simulink model "BimanualCarvingModifiedSnapshot"  (R2013a)
settings: Solver=ode4  SolverMode=SingleTasking  StartTime=0.0  StopTime=inf  FixedStep=0.0005  RelTol=1e-3
StartFcn:
  |  warndlg('Dexterit-E models cannot run under simulation. Please compile your model and run it from within Dexterit-E.');set_param(bdroot,'SimulationCommand','stop')
model workspace (MAT data in the model file):
  BKIN_STEP_TIME = 0.0005
  col_x = 1
  col_y = 2
  WIDTH = 3
  HEIGHT = 4
  TARGET_COL = 1
  LOAD = 2
  TRAJ_DURATION_COL = 3
  MAX_LOAD = 2
  FORCE_ON = 1
  HAND_RADIUS = 6
  REST_COL = 4
  TRAINING_COL = 5
  HAND_COLOR = 5
  TARGET_STROKE = 8
  TARGET_RADIUS = 9
  xMaxCursor = 15
  yMaxCursor = 16
  TARGET_COLOR = 7
  START_X = 10
  START_Y = 11
  STIFFNESS_MATERIAL = 3
  MATERIAL_MASS = 4
  MATERIAL_DAMPING = 5
  STIFFNESS_HANDS = 6
  MATERIAL_GOAL_COLOR = 12
  SCALE_VIBRATION = 7
  STONE_WIDTH = 6
  MATERIAL_DUCTILITY = 8
  TARG_COLOR = 1
  TEXT_COLOR = 13
  TEXTBOX_WIDTH = 14
  TEXTBOX_HEIGHT = 15
  ROTATION = 16
  LABEL_TEXT = 17
  LABEL_COLOR = 18
  LABEL_HEIGHT = 19
  ADVANCE_EMG_PLACEMENT = 2
  ADVANCE_EMG_MAX = 3
  EMG_ADVANCE_BUTTON = 1
  EMG_MVC_BUTTON = 2
  START_TRIAL = 3
  END_TRIAL = 4
  MUSC_NUM = 2
  HAND_DISTANCE = 3
  SYN_NUM = 4
undefined symbols (not defined in the file or in its folder): slselsubs
libraries: xpclib x9, simulink x6, General x3, KINARM_loads x2, Video x2, KINARM_IO x1, KINARM_EP_loads x1
(part 6 of 6)

== matlab function BimanualCarvingModifiedSnapshot/MATLAB Function ==
  data: resid output; emg input; syn_num input
function resid  = emg_similarity(emg,syn_num)
%#codegen

persistent C;

if isempty(C)
    switch syn_num
        case 6
            C = master_synergies_6();
        case 7
            C = master_synergies_7();
        case 8
            C = master_synergies_8();
        case 9
            C = master_synergies_9();
        case 10
            C = master_synergies_10();
        case 11
            C = master_synergies_11();
        case 12
            C = master_synergies_12();
        case 13
            C = master_synergies_13();
        case 14
            C = master_synergies_14();
        case 15
            C = master_synergies_15(); 
        case 16
            C = master_synergies_16();
        otherwise
            C = master_synergies_7();
    end
end

d = emg(1:end,1);

n = size(C,2);
% Initialize vector of n zeros and Infs (to be used later)
nZeros = zeros(n,1);
wz = nZeros;

% Initialize set of non-active columns to null
P = false(n,1);
% Initialize set of active columns to all and the initial point to zeros
Z = true(n,1);
x = nZeros;

resid = d - C*x;
w = C'*resid;

% Set up iteration criterion
outeriter = 0;
iter = 0;
itmax = 3*n;

tol = 10*eps*norm(C,1)*length(C);

% Outer loop to put variables into set to hold positive coefficients
while any(Z) && any(w(Z) > tol)
    outeriter = outeriter + 1;
    % Reset intermediate solution z
    z = nZeros;
    % Create wz, a Lagrange multiplier vector of variables in the zero set.
    % wz must have the same size as w to preserve the correct indices, so
    % set multipliers to -Inf for variables outside of the zero set.
    wz(P) = -Inf;
    wz(Z) = w(Z);
    % Find variable with largest Lagrange multiplier
    [~,t] = max(wz);
    % Move variable t from zero set to positive set
    P(t) = true;
    Z(t) = false;
    % Compute intermediate solution using only variables in positive set
    z(P) = C(:,P)\d;
    % inner loop to remove elements from the positive set which no longer belong
    while any(z(P) <= 0)
        iter = iter + 1;
        if iter > itmax
            %            msg = getString(message('MATLAB:lsqnonneg:IterationCountExceeded'));
            %            if verbosity
            %                disp(msg)
            %            end
            %            exitflag = 0;
            %            output.iterations = outeriter;
            %            output.message = msg;
            %            output.algorithm = 'active-set';
            resnorm = sum(resid.*resid);
            x = z;
            lambda = w;
            return
        end
        % Find indices where intermediate solution z is approximately negative
        Q = (z <= 0) & P;
        % Choose new x subject to keeping new x nonnegative
        alpha = min(x(Q)./(x(Q) - z(Q)));
        x = x + alpha*(z - x);
        % Reset Z and P given intermediate values of x
        Z = ((abs(x) < tol) & P) | Z;
        P = ~Z;
        z = nZeros;           % Reset z
        z(P) = C(:,P)\d;      % Re-solve for z
    end
    x = z;
    resid = d - C*x;
    w = C'*resid;
end
end

function C = master_synergies_6()

C = [ 0.6059         0    0.0982    0.3257    0.0587    0.0562;
    0.3321    0.1853    0.0774    0.0907    0.3019    0.1813;
    0.1383    0.6018         0    0.1365         0    0.2733;
    0    0.0039    0.4293    0.0680    0.2207         0;
    0.1053    0.4074         0         0         0    0.2375;
    0.1749         0    0.7674    0.1333    0.0094    0.1202;
    0.2135    0.4062         0    0.0447    0.0003    0.0525;
    0.3188         0    0.2392    0.0240    0.3338         0;
    0.2886         0         0    0.5969    0.0171    0.3358;
    0.0632    0.0389    0.0341    0.0191    0.2286    0.4584;
    0.2456    0.0036    0.3484    0.4769    0.6912         0;
    0.0068    0.4849    0.0629    0.3820    0.1736    0.1716;
    0.1126    0.0665    0.1033    0.2344    0.4184    0.0828;
    0    0.0880         0    0.1599         0    0.5841;
    0.2590    0.1541    0.1131    0.1704         0    0.1773;
    0.2953    0.0010    0.0630    0.0508    0.0982    0.2895];
end

function C = master_synergies_7()

C = [0.2361    0.5046    0.0063    0.0514    0.0762    0.1018    0.5583;
    0.0626    0.6381    0.2251    0.0416    0.0042    0.3024    0.1665;
    0.0099    0.1110    0.0041    0.5932    0.0038    0.2818    0.0222;
    0.3413         0    0.3384         0    0.0118         0    0.0002;
    0    0.1591         0    0.3446         0    0.2055         0;
    0.8267    0.0618    0.2096    0.0154    0.0543    0.1097    0.0277;
    0.0486    0.0867         0    0.4538    0.2466         0    0.0104;
    0.2047    0.3779    0.3780         0    0.1608         0    0.0902;
    0.0667    0.0003    0.0100    0.1339    0.1139    0.4125    0.5722;
    0    0.0064    0.0628         0    0.6909    0.2578         0;
    0.2141    0.2612    0.6779    0.0381    0.1927    0.1565    0.4705;
    0.0114    0.0040    0.2441    0.5000    0.0084    0.3172    0.1190;
    0.0198    0.1710    0.3527    0.0473    0.1981    0.1708    0.2149;
    0.0064    0.0110    0.0010    0.0279    0.0479    0.5863         0;
    0.1867    0.0999    0.0025    0.2151    0.2154    0.1211    0.1699;
    0.1015    0.1971    0.0198    0.0118    0.5375    0.1232    0.1141];

end

function C = master_synergies_8()

C = [ 0.4473    0.3964    0.1653    0.0355    0.1020    0.5229    0.0261    0.0115;
    0.0285    0.7249    0.0686    0.0500    0.0628    0.2279    0.0889    0.3301;
    0.0517    0.0993    0.1484    0.6898    0.3641    0.0000    0.0003    0.0000;
    0.0250    0.0000    0.0000    0.0000    0.0000    0.0867    0.4422    0.1256;
    0.0000    0.1156    0.0027    0.4693    0.2537    0.0006    0.0000    0.0081;
    0.0285    0.0118    0.0145    0.0000    0.1628    0.3434    0.7008    0.0000;
    0.0281    0.0338    0.4232    0.4431    0.0439    0.1244    0.0000    0.0362;
    0.1715    0.0510    0.0000    0.0856    0.0000    0.5682    0.1402    0.2302;
    0.5959    0.0444    0.1387    0.0688    0.5056    0.0768    0.0286    0.0373;
    0.0052    0.0000    0.0548    0.0259    0.2395    0.0613    0.0407    0.5230;
    0.5523    0.3729    0.0916    0.0230    0.0091    0.0773    0.4871    0.5104;
    0.0226    0.2717    0.8393    0.1750    0.2185    0.0406    0.0678    0.1765;
    0.2321    0.2706    0.0940    0.0305    0.0456    0.0082    0.1862    0.3985;
    0.0000    0.0440    0.0002    0.0000    0.5584    0.0000    0.0000    0.1577;
    0.1892    0.0177    0.1459    0.2290    0.2196    0.2362    0.0772    0.0182;
    0.1200    0.0002    0.0386    0.0810    0.1930    0.3711    0.0000    0.2650];

end

function C = master_synergies_9()

C = [0.4154    0.1071    0.1031    0.5616         0    0.0589    0.1282         0    0.1961;
    0.2289    0.0221    0.0624    0.6351    0.0007         0    0.3077    0.2958         0;
    0.0457         0    0.3796    0.1022    0.7570    0.2097    0.0499         0         0;
    0.0908    0.4127         0         0         0    0.0101    0.1940    0.0988         0;
    0         0    0.2481    0.0969    0.5721         0    0.1394    0.0069         0;
    0.0770    0.8327    0.0579    0.1964         0         0    0.0150    0.0748    0.1636;
    0         0    0.0124    0.2192    0.2617    0.4170         0         0    0.4660;
    0.1660    0.1223         0    0.2036         0         0    0.6855         0    0.1629;
    0.4004         0    0.5906    0.0466    0.0589    0.1919    0.1056         0         0;
    0.0041         0    0.0842         0    0.0131         0    0.0481    0.6103    0.5818;
    0.6728    0.3045    0.0577    0.1792         0    0.0962    0.2672    0.4640         0;
    0.0379         0    0.3971    0.1856         0    0.8413    0.3095    0.0652         0;
    0.3270    0.0679    0.0566    0.1250    0.0255    0.0633    0.1523    0.3976    0.0374;
    0         0    0.4330    0.1048    0.0002    0.0136    0.0168    0.3790         0;
    0.0968    0.1093    0.2007    0.1583    0.1635    0.1432    0.0970         0    0.2817;
    0.0220         0    0.1686    0.1138    0.0077         0    0.3817    0.0579    0.5213];
end

function C = master_synergies_10()

C = [0.4986    0.1733    0.0367    0.4603    0.1482         0    0.0499    0.0111    0.0009         0;
    0.5610    0.0771    0.2267         0    0.0812    0.0400         0    0.5313         0         0;
    0         0    0.6666    0.1875    0.1703         0         0    0.1027    0.5281    0.1122;
    0    0.3723         0         0         0    0.2823         0         0    0.0324    0.3422;
    0.0393         0    0.5953    0.0003    0.0925         0    0.1203    0.0059    0.1207    0.0717;
    0    0.8366    0.0060    0.0965    0.0166    0.2299    0.0212    0.0633    0.0647    0.2363;
    0.0961         0    0.1922    0.0963    0.1991         0    0.0015    0.0222    0.7730    0.0491;
    0.4351    0.0715         0         0         0    0.0157    0.0037    0.0915         0    0.7138;
    0.0336         0    0.0213    0.7040    0.2206    0.1786    0.2542    0.1029         0    0.2509;
    0         0         0    0.0018         0    0.2589    0.6350    0.2435    0.1760    0.0651;
    0.3789    0.3157         0    0.3611    0.1261    0.7676    0.1259         0    0.0010    0.1354;
    0.1213         0    0.2816    0.0028    0.8945         0    0.3734    0.0095         0    0.1218;
    0.2207    0.0857    0.0583    0.1355    0.1095    0.4212    0.2106    0.0735         0         0;
    0         0    0.0758    0.0610    0.0479    0.0076    0.1904    0.7866    0.0100    0.0738;
    0.0641    0.1157    0.1403    0.2653    0.1074    0.0026    0.1498         0    0.2697    0.2213;
    0.1560         0    0.0542    0.1260    0.0596         0    0.5065         0         0    0.3776];

end

function C = master_synergies_11()

C = [ 0.6267         0         0    0.3526         0    0.5868         0    0.0290         0    0.0100         0;
    0.0928         0    0.2848    0.7848         0    0.2838         0         0    0.1110         0         0;
    0.0727    0.7087    0.0213    0.0284         0    0.0469    0.1440         0    0.2549    0.4188         0;
    0         0    0.3660         0    0.3437         0         0    0.0812    0.0430    0.0288    0.0164;
    0    0.5699         0    0.0503    0.0029    0.1112         0    0.0926    0.1385         0    0.0129;
    0.2034         0    0.1110    0.1557    0.9149    0.0419    0.0453    0.1059    0.0242    0.0716         0;
    0.0633    0.2088         0    0.1548         0    0.1978         0         0    0.0780    0.8336    0.1164;
    0         0    0.5202    0.0670         0    0.5700         0         0    0.2355    0.0045    0.0189;
    0.4181    0.0649    0.0571    0.0372         0         0    0.3762    0.0922    0.6754         0         0;
    0.0004         0         0         0    0.0498    0.1478    0.3393    0.6502    0.0067    0.2170         0;
    0.5158         0    0.6441    0.2784    0.0183    0.1438         0    0.4946         0         0         0;
    0.1802    0.3229         0    0.2333         0    0.1151    0.2538         0         0         0    0.9915;
    0.2333    0.0377    0.2887    0.2184         0    0.0854    0.0204    0.3955         0         0    0.0446;
    0    0.0579    0.0068    0.0512    0.0187         0    0.8089         0    0.1247    0.0439    0.0094;
    0.1421    0.1273         0    0.1116    0.1612    0.1440    0.0371    0.0738    0.3545    0.2731         0;
    0         0         0    0.0872    0.1255    0.3331         0    0.3674    0.4921    0.0055    0.0246];

end

function C = master_synergies_12()

C = [ 0.7011         0    0.1260         0    0.4795         0    0.0246    0.1420         0         0    0.2258       0;
    0.2721         0    0.0341         0    0.3797    0.2816    0.5681    0.2077         0         0         0    0.3002;
    0         0    0.2804         0    0.0110    0.3023         0    0.4993    0.1884    0.2485    0.0360    0.9492;
    0    0.4017         0    0.4368    0.0518         0    0.0317         0         0         0         0         0;
    0    0.0125    0.1436         0         0    0.1829         0    0.7672    0.0852    0.1739    0.0414    0.0511;
    0.1513    0.8869         0    0.2600    0.0407    0.0063    0.0048         0    0.0045    0.0497    0.1281    0.0421;
    0.0491         0    0.7884         0    0.0348    0.0997         0    0.0379    0.0678    0.2205    0.0185    0.0169;
    0.1555         0         0    0.4127    0.6706         0    0.0501    0.0471    0.0002         0    0.0063         0;
    0.2981         0    0.0862    0.1803    0.0589    0.4909    0.0959         0    0.0596    0.5564         0    0.0600;
    0.0326         0    0.0000    0.0327    0.0957         0    0.2165         0         0    0.1787    0.8417         0;
    0.4802    0.1772    0.0091    0.6794    0.2152         0    0.5173    0.0512    0.0034         0    0.2337         0;
    0    0.0120    0.3977         0    0.0096    0.2549    0.2803    0.2526    0.9724         0    0.0483    0.0023;
    0.2241    0.0102         0    0.2667    0.1009    0.0233    0.4269    0.1000    0.0537    0.0253    0.2408    0.0237;
    0    0.0279    0.0178    0.0066         0    0.6702         0    0.0787    0.0074    0.0318    0.2909         0;
    0.1181    0.1386    0.3100    0.0703    0.0903    0.1730    0.0262    0.1014         0    0.3897         0         0;
    0.0119    0.0145         0         0    0.3052    0.0156    0.2964    0.0471    0.0229    0.6015    0.1454         0];

end

function C = master_synergies_13()

C = [0.4192    0.0916         0         0         0    0.0643    0.3018    0.9064         0         0    0.1337    0.0079         0;
    0.3740    0.1303         0    0.1148         0         0    0.0495         0    0.2485         0    0.9012         0    0.0689;
    0.0322    0.7385         0    0.1716    0.3918    0.1511    0.1826         0    0.0703         0         0         0    0.1042;
    0.0513         0    0.3098    0.0162         0    0.0250    0.2180    0.0287         0    0.4563    0.1158         0    0.0011;
    0    0.5836         0         0         0         0    0.0697    0.0258    0.2212         0    0.1315    0.2304    0.1023;
    0.2294         0    0.9350    0.0655    0.0864    0.1329    0.0127    0.1139         0    0.0007    0.0609         0    0.0907;
    0.0489    0.2372         0         0    0.7054         0    0.2310    0.1142         0         0    0.1122    0.1288    0.0107;
    0.3397         0         0         0         0    0.0715    0.7998    0.1187    0.0394         0         0    0.0459    0.1225;
    0.1882    0.0494         0    0.3749    0.1292    0.7747    0.0972    0.0989         0         0    0.1000         0    0.0593;
    0.0007         0    0.0600    0.1048    0.0239    0.0557    0.0621    0.0192         0         0    0.1753    0.3761    0.8602;
    0.5917         0    0.1283    0.0382    0.0683    0.3674    0.0732    0.2509         0    0.7505         0         0    0.3835;
    0.0010         0    0.0467    0.3337    0.5202    0.3822         0    0.1442    0.9369         0         0    0.0102         0;
    0.2740    0.0167         0    0.0743    0.0172    0.1146         0    0.1462    0.0711    0.4782    0.1199    0.1512    0.2451;
    0    0.0189    0.0160    0.8255    0.0421    0.0019    0.0789         0    0.0051         0    0.0309    0.0256         0;
    0.0777    0.1713    0.0859    0.0264    0.2161    0.2037    0.2027    0.1422         0         0    0.2586    0.2396         0;
    0.2087         0         0    0.0272    0.0044    0.1032    0.2481    0.0356         0         0         0    0.8400         0];

end

function C = master_synergies_14()

C = [0.0658    0.8315    0.3623    0.3054    0.0918         0    0.0154         0         0    0.1063         0         0         0    0.0079;
    0.0038    0.3625         0    0.1597    0.8230         0         0    0.1820         0         0         0         0    0.1647    0.1061;
    0    0.0541    0.2498    0.1010    0.0496         0    0.1656    0.5613    0.8729    0.0257    0.1291         0         0    0.0075;
    0.1531    0.0414    0.0043    0.0970    0.0583    0.1241         0         0         0    0.0125    0.0395         0    0.8465    0.0420;
    0         0    0.1842         0         0         0    0.0825    0.7553    0.1601    0.0338    0.0950    0.1002         0    0.0899;
    0.1360    0.0882    0.1645    0.1577    0.0862    0.9568         0         0         0         0         0         0    0.4057    0.1042;
    0    0.1579    0.1105    0.1048         0         0         0    0.1761    0.3970    0.0331    0.0056         0         0    0.9063;
    0.0668    0.2608         0    0.6901    0.1444    0.0418         0         0         0    0.1791         0         0    0.1005         0;
    0.2427    0.0194    0.7816    0.2601    0.1676         0    0.0265         0         0    0.1390    0.0530         0         0    0.0048;
    0.0105         0         0    0.1403    0.1383    0.0058    0.0034    0.0184    0.0012    0.1897    0.1011    0.9044         0    0.0034;
    0.8485    0.1839    0.1112    0.4146    0.3034    0.2377         0         0         0    0.2042    0.1958         0         0    0.0351;
    0.0438    0.0806    0.0721    0.1096         0         0    0.9805    0.1726    0.1986    0.1481         0    0.3109         0    0.2030;
    0.4103    0.1052         0    0.1103    0.2762         0    0.0534    0.0558    0.0098    0.2449    0.1476    0.1096    0.0880         0;
    0         0    0.0426    0.0213    0.1013         0    0.0247    0.0316    0.0256    0.0593    0.9484    0.2518    0.0582    0.0128;
    0    0.1418    0.3207    0.1245    0.0900    0.0485         0    0.1266    0.1211    0.1976         0         0    0.2632    0.3220;
    0.0021    0.0079    0.0009    0.2240    0.2149    0.0923    0.0058         0         0    0.8556    0.0127         0    0.0364    0.0132];

end

function C = master_synergies_15()

C = [ 0.4462    0.7696         0    0.2903         0         0    0.0693         0         0    0.0006         0         0    0.0000    0.0118         0;
    0.3767    0.3395         0         0    0.0120         0         0    0.0207    0.0371    0.9074         0         0         0    0.2974         0;
    0    0.0040    0.8797         0         0    0.1721    0.3340         0    0.2984    0.1297    0.0427    0.1668         0         0         0;
    0.1327         0         0    0.2290    0.1006         0    0.0137         0    0.1129    0.0016         0         0    0.0679         0    0.9196;
    0    0.0073    0.2200         0         0    0.0807    0.0798    0.0457    0.1362    0.0635    0.0912    0.9854    0.0051    0.0026         0;
    0.1486         0         0    0.8910    0.1577    0.0458    0.0438    0.0021    0.2191    0.1773    0.0140         0    0.1226         0    0.2379;
    0    0.1039    0.2719    0.0030         0    0.0000    0.0271    0.0300    0.3131    0.0585         0         0    0.9676    0.0232         0;
    0.6055    0.0611         0    0.0793         0         0    0.0546    0.0100         0    0.0382         0    0.0278    0.1488    0.2845    0.2191;
    0    0.2531         0         0         0    0.8757    0.4786         0         0    0.3254         0         0         0         0    0.1597;
    0.0216    0.0185         0         0         0    0.2234    0.0357    0.0014    0.0722         0    0.9429         0    0.0137    0.2560    0.0295;
    0.4505    0.3196         0    0.1866    0.8805    0.1448    0.1148         0         0    0.0057         0         0    0.0381    0.0827         0;
    0.0003    0.2049    0.3036         0         0    0.0970         0    0.9966    0.2444    0.0934    0.0205         0    0.0080    0.1401         0;
    0.1447    0.2373    0.0215    0.0175    0.4355    0.0617    0.0844    0.0412         0    0.0509    0.0855         0         0    0.2367    0.1230;
    0.0025         0    0.0105         0         0         0    0.7774    0.0396    0.0906    0.0457    0.3043    0.0173    0.0268    0.0606    0.0274;
    0.1669    0.1120    0.1050    0.0431         0    0.1324         0         0    0.7851    0.0133    0.0150         0    0.0779         0    0.0744;
    0.0230    0.0211         0    0.1616         0    0.3054    0.1286    0.0031    0.2069         0         0         0    0.1162    0.8235    0.0445];

end

function C = master_synergies_16()

C = [0.0000    1.0000         0         0         0    0.0000    0.0000    0.0000    0.0000    0.0000    0.0000         0    0.0000    0.0000    0.0000         0;
    0         0         0    0.0000         0    0.0000    1.0000         0    0.0000    0.0000    0.0000    0.0000    0.0000    0.0000         0         0;
    0    0.0000         0    0.0000    1.0000    0.0000         0    0.0000         0         0         0    0.0000    0.0000    0.0000    0.0000    0.0000;
    0    0.0000         0         0    0.0000    0.0000    0.0000         0         0    0.0000         0         0    0.0000    0.0000         0    1.0000;
    0.0000    0.0000    0.0000    0.0000         0    0.0000    0.0000    0.0000    0.0000         0         0    1.0000    0.0000    0.0000         0         0;
    0.0000         0    0.0000    1.0000         0    0.0000    0.0000         0    0.0000         0    0.0000    0.0000    0.0000    0.0000         0    0.0000;
    0.0000    0.0000         0         0    0.0000    0.0000         0    0.0000    0.0000    1.0000    0.0000    0.0000    0.0000         0         0         0;
    0.0000         0         0    0.0000    0.0000    0.0000         0    1.0000    0.0000    0.0000    0.0000         0         0         0    0.0000         0;
    0.0000    0.0000    0.0000    0.0000         0    1.0000    0.0000         0    0.0000         0    0.0000         0         0    0.0000    0.0000    0.0000;
    0.0000         0    0.0000         0    0.0000    0.0000         0    0.0000    0.0000    0.0000    0.0000    0.0000         0    1.0000         0         0;
    1.0000    0.0000    0.0000         0         0    0.0000         0         0    0.0000    0.0000    0.0000    0.0000    0.0000    0.0000         0         0;
    0    0.0000    1.0000    0.0000    0.0000    0.0000         0    0.0000    0.0000         0    0.0000         0         0    0.0000    0.0000    0.0000;
    0    0.0000    0.0000    0.0000    0.0000    0.0000    0.0000         0    1.0000    0.0000    0.0000         0    0.0000    0.0000         0    0.0000;
    0.0000    0.0000    0.0000    0.0000         0    0.0000    0.0000    0.0000         0    0.0000    0.0000         0    0.0000         0    1.0000    0.0000;
    0.0000         0    0.0000    0.0000    0.0000         0         0         0    0.0000    0.0000    1.0000         0    0.0000    0.0000    0.0000    0.0000;
    0    0.0000    0.0000    0.0000         0         0         0         0         0    0.0000    0.0000    0.0000    1.0000    0.0000    0.0000         0];

end
